simulink model "ControladorCorriente"  (R2026b)
settings: Solver=VariableStepAuto
values from neighbouring files (symbols this model uses):
  i_m_max = 5    [Pendulo_Invertido.m]
  i_m_min = -i_m_max    (= -5)    [Pendulo_Invertido.m]
  Ki_i = Ra*omega_i    (= 288.5)    [Pendulo_Invertido.m]
  Kp_i = La*omega_i    (= 0.0955)    [Pendulo_Invertido.m]
  v_max = 24    [Pendulo_Invertido.m]
  v_min = -v_max    (= -24)    [Pendulo_Invertido.m]
libraries: eeGeneralControl x1
settings Model: Creator=fedeb  LastModifiedBy=fedeb

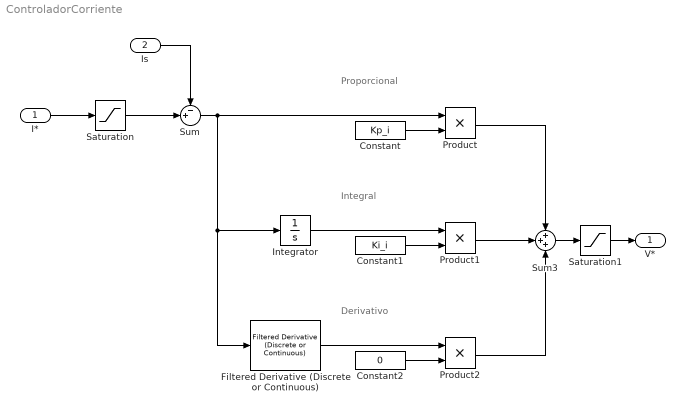
== system ControladorCorriente ==
  note: Proporcional
  note: Integral
  note: Derivativo
  Ⅰ* : Inport
  Ⅰs : Inport  Port=2
  Constant : Constant  Value=Kp_i
  Constant1 : Constant  Value=Ki_i
  Constant2 : Constant  Value=0
  Filtered Derivative (Discrete or Continuous) : eeGeneralControl/Filtered Derivative (Discrete or Continuous)  K=1  T=0.1  B=inf  A=-inf  minRatio=10  init_option=Specify as parameter  x0=i_init  Ts=-1
      settings: LibrarySourceBlock=|
      | ee_sl_lib/General Control/Filtered Derivative
      | (Discrete or Continuous)
  Integrator : Integrator
  Product : Product
  Product1 : Product
  Product2 : Product
  Saturation : Saturate  UpperLimit=i_m_max  LowerLimit=i_m_min
  Saturation1 : Saturate  UpperLimit=v_max  LowerLimit=v_min
  Sum : Sum  Inputs=-+|
  Sum3 : Sum  Inputs=+++
  V* : Outport
  wires:
  Ⅰs/1 -> Sum/1
  Product/1 -> Sum3/1
  Constant/1 -> Product/2
  Sum3/1 -> Saturation1/1
  Sum/1 -> Integrator/1, Filtered Derivative (Discrete or Continuous)/1, Product/1
  Constant1/1 -> Product1/2
  Integrator/1 -> Product1/1
  Filtered Derivative (Discrete or Continuous)/1 -> Product2/1
  Constant2/1 -> Product2/2
  Product1/1 -> Sum3/2
  Product2/1 -> Sum3/3
  Ⅰ*/1 -> Saturation/1
  Saturation/1 -> Sum/2
  Saturation1/1 -> V*/1
